simulink model "detecteur_optimal"  (R2023b)
settings: Solver=FixedStepDiscrete  StartTime=0.0  StopTime=N*Tb - Te  FixedStep=Te  RelTol=1e-3
values from neighbouring files (symbols this model uses):
  A = P.A    [parametres.m]    (also in partie2_1.m; partie2_5_q10.m = numel(unique(msg)); partie2_5_q11.m = numel(unique(seq)))
  graine = P.graine    [parametres.m]    (also in parametres_perso.m = mod(sum(c .* (1:numel(c)) * 31) + 7 * numel(c), 2^31 - 1); partie2_1.m)
  L = P.L    [parametres.m]    (also in partie2_1.m)
  sig2 = N0 * L / (2*Tb)    [parametres.m]    (also in partie3_q12.m = A^2 * L / (2 * 10^(EbN0dB/10)))
  Tb = 1    [parametres.m]    (also in partie2_1.m)
  Te = 1/Lq    [lancer.m]    (also in lancer_echo.m; parametres.m = Tb / L)
libraries: simulink x3
settings Model: Creator=e2507477  LastModifiedBy=e2507477

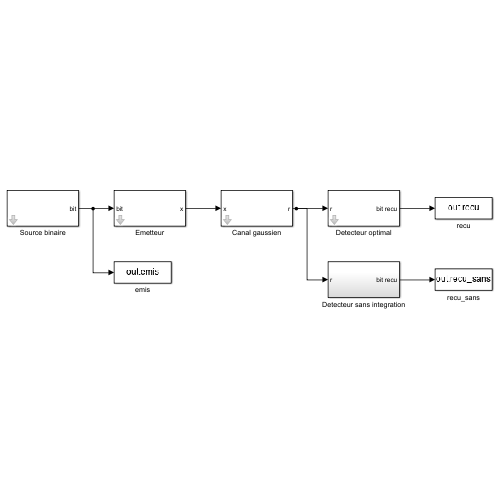
[thumbnail: Simulink's stored preview of the top-level diagram]
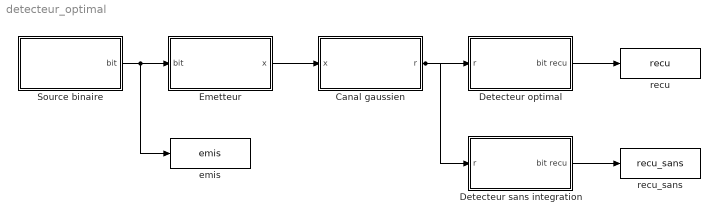
== system detecteur_optimal ==
  Canal gaussien : Subsystem  mask{sig2=sig2, Te=Te, graine=graine}
      mask prompts: sig2 "Variance par échantillon"
  Detecteur optimal : Subsystem  mask{L=L, Te=Te, Tb=Tb}
      mask prompts: L "Échantillons par bit L"
  Detecteur sans integration : Subsystem
  Emetteur : Subsystem  mask{A=A, Te=Te}
      mask prompts: A "Amplitude A"; Te "Période d'échantillonnage Te"
  Source binaire : Subsystem  mask{p1=0.5, Tb=Tb, graine=graine}
      mask prompts: p1 "Probabilité d'un 1"; Tb "Durée d'un bit"
  emis : ToWorkspace  VariableName=emis  SampleTime=-1
  recu : ToWorkspace  VariableName=recu  SampleTime=-1
  recu_sans : ToWorkspace  VariableName=recu_sans  SampleTime=-1
  wires:
  Source binaire/1(bit) -> Emetteur/1(bit), emis/1
  Emetteur/1(x) -> Canal gaussien/1(x)
  Canal gaussien/1(r) -> Detecteur optimal/1(r), Detecteur sans integration/1(r)
  Detecteur optimal/1(bit recu) -> recu/1
  Detecteur sans integration/1(bit recu) -> recu_sans/1

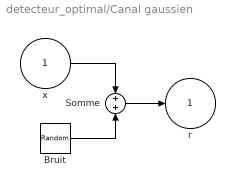
== system detecteur_optimal/Canal gaussien ==
  x : Inport
  Bruit : RandomNumber  Variance=sig2  Seed=round(graine)+5000  SampleTime=Te
  Somme : Sum
  r : Outport
  wires:
  Bruit/1 -> Somme/2
  x/1 -> Somme/1
  Somme/1 -> r/1

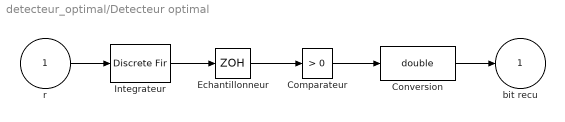
== system detecteur_optimal/Detecteur optimal ==
  r : Inport
  Comparateur : simulink/Logic and Bit Operations/Compare To Constant  relop=>  const=0  OutDataTypeStr=boolean
  Conversion : DataTypeConversion  OutDataTypeStr=double  SaturateOnIntegerOverflow=off  RndMeth=Floor
  Echantillonneur : ZeroOrderHold  SampleTime=[Tb (L-1)*Te]
  Integrateur : DiscreteFir  Coefficients=ones(1,L)/L  SampleTime=Te
  bit recu : Outport
  wires:
  r/1 -> Integrateur/1
  Conversion/1 -> bit recu/1
  Comparateur/1 -> Conversion/1
  Integrateur/1 -> Echantillonneur/1
  Echantillonneur/1 -> Comparateur/1

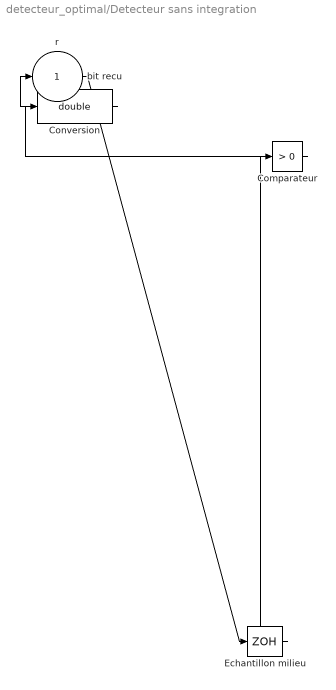
== system detecteur_optimal/Detecteur sans integration ==
  r : Inport
  Comparateur : simulink/Logic and Bit Operations/Compare To Constant  relop=>  const=0  OutDataTypeStr=boolean
  Conversion : DataTypeConversion  OutDataTypeStr=double  SaturateOnIntegerOverflow=off  RndMeth=Floor
  Echantillon milieu : ZeroOrderHold  SampleTime=[Tb floor(L/2)*Te]
  bit recu : Outport
  wires:
  r/1 -> Echantillon milieu/1
  Echantillon milieu/1 -> Comparateur/1
  Comparateur/1 -> Conversion/1
  Conversion/1 -> bit recu/1

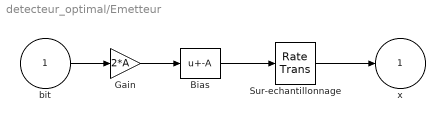
== system detecteur_optimal/Emetteur ==
  bit : Inport
  Bias : Bias  Bias=-A  SaturateOnIntegerOverflow=off
  Gain : Gain  Gain=2*A
  Sur-echantillonnage : RateTransition  OutPortSampleTime=Te
  x : Outport
  wires:
  bit/1 -> Gain/1
  Gain/1 -> Bias/1
  Bias/1 -> Sur-echantillonnage/1
  Sur-echantillonnage/1 -> x/1

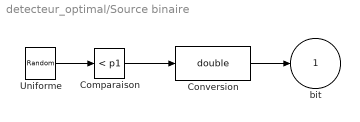
== system detecteur_optimal/Source binaire ==
  Comparaison : simulink/Logic and Bit Operations/Compare To Constant  relop=<  const=p1  OutDataTypeStr=boolean
  Conversion : DataTypeConversion  OutDataTypeStr=double  SaturateOnIntegerOverflow=off  RndMeth=Floor
  Uniforme : UniformRandomNumber  Minimum=0  Seed=round(graine)  SampleTime=Tb
  bit : Outport
  wires:
  Uniforme/1 -> Comparaison/1
  Comparaison/1 -> Conversion/1
  Conversion/1 -> bit/1
